simulink model "pakmpc_rw_combined"  (R2026b)
settings: Solver=ode45  StopTime=200  MaxStep=0.01  RelTol=1e-8  AbsTol=1e-10
values from neighbouring files (symbols this model uses):
  m = @(x) mat2str(x, 17)    [build_combined_multibody.m]    (also in build_pakmpc_multibody.m)
  s = q(1)    [build_combined_multibody.m]    (also in build_pakmpc_multibody.m; build_rw_array.m = runcheck(mdl, r4, [1 0 0 0], [0 0 0], u4, 0, 5))
undefined symbols (not defined in the file or in its folder): DiscIntNeverNeededParam, X, Y, Z
libraries: sm_lib x58, nesl_utility x12
(part 2 of 2)

== matlab function pakmpc_rw_combined/RW Allocation ==
  data: u input; mm output; dw input; p input
function mm = alloc(u, dw, p)
% Maps desired 3-axis torque u into 4 tetrahedral wheels: M_m = -W_T^+ u - dw
u = u(:); dw = dw(:); p = p(:);
wp = [0.61237243569579436 0.43301270189221919 0;-0.61237243569579436 0.43301270189221924 0;0 0.43301270189221935 0.61237243569579436;0 0.43301270189221935 -0.61237243569579436];
jw = 0.080000000000000002; taumax = 0.5; hmax = 50;
mm = -wp*u - dw;
mm = min(max(mm, -taumax), taumax);
mm(abs(jw*p) >= hmax & sign(mm) == sign(p)) = 0;

== matlab function pakmpc_rw_combined/Target Torque ==
  data: q input; ut output; w input
function ut = target(q, w)
q = q(:); w = w(:);
a = [0.5;-0.5;-0.5;-0.5];
kpt = [0.73599999999999999 0 0;0 0.75 0;0 0 0.73599999999999999]; kdt = [1.8399999999999999 0 0;0 1.875 0;0 0 1.8399999999999999];
qv = a(1)*q(2:4) + q(1)*a(2:4) + cross(a(2:4), q(2:4));
ut = -kpt*qv - kdt*w;

== matlab function pakmpc_rw_combined/Disturbance ==
  data: t input; td output
function td = dist(t)
td = [0.1*sin(0.075*t); -0.2*sin(0.1*t); 0.15*sin(0.1*t)];
